simulink model "Encoder_1"  (R2020a)
settings: Solver=FixedStepAuto  StartTime=0.0  StopTime=inf  RelTol=1e-3  EnableMultiTasking=on
libraries: mkrmotorcarrierlib x1, eeGeneralControl x1
settings Model: SILPILModeSetting=veronly  ExtModeTrigDuration=2  Creator=bkhusain  LastModifiedBy=mmarathe
settings OptimizationCC: EnhancedBackFolding=on  PassReuseOutputArgsAs=Individual arguments  ZeroExternalMemoryAtStartup=off  ZeroInternalMemoryAtStartup=off  MaxStackSize=64  OptimizeBlockOrder=speed  DifferentSizesBufferReuse=on  OptimizationCustomize=off  EfficientTunableParamExpr=on
settings DebuggingCC: ParameterTunabilityLossMsg=error
settings HardwareCC: ProdBitPerPointer=32  ProdBitPerSizeT=32  ProdBitPerPtrDiffT=32  ProdLargestAtomicInteger=Long  ProdLargestAtomicFloat=Double  ProdWordSize=32  ProdHWDeviceType=ARM Compatible->ARM Cortex
settings SFSimCC: MATLABDynamicMemAlloc=off
settings RTWCC: SystemTargetFile=ert.tlc  HardwareBoard=Arduino Nano 33 IoT  TLCOptions=-aInlineSetEventsForThisBaseRateFcn=TLC_FALSE -aSuppressMultiTaskScheduler=TLC_FALSE -aRateBasedStepFcn=1  TemplateMakefile=ert_default_tmf  Toolchain=Arduino ARM  BuildConfiguration=Faster Runs
settings CodeAppCC: ForceParamTrailComments=on  IgnoreCustomStorageClasses=off  OperatorAnnotations=on  SimulinkDataObjDesc=on  SFDataObjDesc=on  InsertBlockDesc=on
settings ERTTargetCC: SupportContinuousTime=on  SupportVariableSizeSignals=on  ExtModeStaticAllocSize=8192

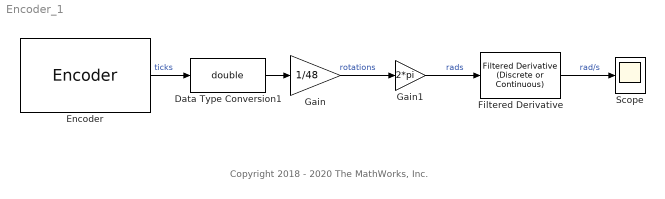
== system Encoder_1 ==
  note: Copyright 2018 - 2020 The MathWorks, Inc.
  Data Type Conversion1 : DataTypeConversion  OutDataTypeStr=double
  Encoder : mkrmotorcarrierlib/Encoder  SlaveAddress=uint8( hex2dec( '66' ) )  blockPlatform=ARDUINO  Encoder=1  ShowSpeed=off  ResetOption=on  SampleTime=0.01
      settings: SourceProductName=Simulink Support for Arduino MKR Motor Carrier
  "Filtered Derivative " : eeGeneralControl/Filtered Derivative (Discrete or Continuous)  K=1  T=0.1  B=inf  A=-inf  minRatio=10  init_option=Inherited from block input  x0=0  Ts=0.01
      settings: SourceProductBaseCode=PS
  Gain : Gain  Gain=1/48
  Gain1 : Gain  Gain=2*pi
  Scope : Scope
  wires:
  Encoder/1 -> Data Type Conversion1/1  "ticks"
  Gain1/1 -> "Filtered Derivative "/1  "rads"
  Data Type Conversion1/1 -> Gain/1
  Gain/1 -> Gain1/1  "rotations"
  "Filtered Derivative "/1 -> Scope/1  "rad/s"
